simulink model "latLinSim"  (R2021b)
settings: Solver=VariableStepAuto  StartTime=0.0  StopTime=20  RelTol=1e-3
values from neighbouring files (symbols this model uses):
  g = 32.17405    [SingleDOF.m]    (also in layer1atm.m; mainSimple.m = 32.174; simio.m = [dx(Index.EOM(1:6)); delta(:)-f; -delta(:)-f ])
  K_lat_hinf = pss(K_lat_hinfs,Domain)    [SingleDOF.m]    (also in latTest.m; main.m; mainSimple.m; test.m)
  LTI_lat = ss(A_lat,B_lat,C_lat,D_lat)    [Dorobantu.m]    (also in mainLinear.m = GTM_lat(:,:,i,j,k))
libraries: simulink_extras x9
settings Model: Creator=jihoo  LastModifiedBy=jihoo

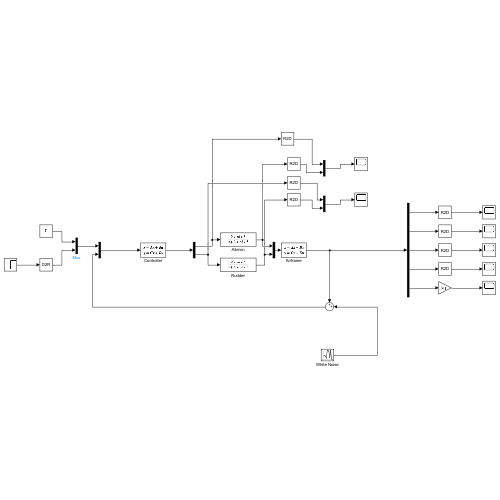
[thumbnail: Simulink's stored preview of the top-level diagram]
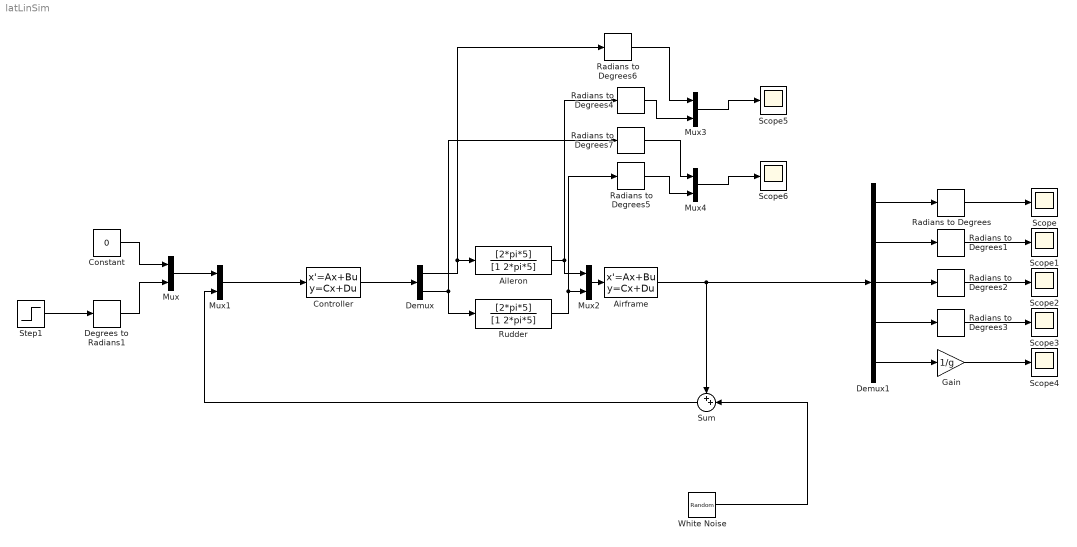
== system latLinSim ==
  Aileron : TransferFcn  Numerator=[2*pi*5]  Denominator=[1 2*pi*5]
  Airframe : StateSpace  A=LTI_lat.A  B=LTI_lat.B  C=LTI_lat.C  D=LTI_lat.D  InitialCondition=0
  Constant : Constant  Value=0
  Controller : StateSpace  A=K_lat_hinf.A  B=K_lat_hinf.B  C=K_lat_hinf.C  D=K_lat_hinf.D  InitialCondition=0
  Degrees to Radians1 : simulink_extras/Transformations/Degrees to Radians
  Demux : Demux  Outputs=2
  Demux1 : Demux  Outputs=5
  Gain : Gain  Gain=1/g
  Mux{,1..4} (5 alike) : Mux  Inputs=2
  Radians to Degrees{,1..7} (8 alike) : simulink_extras/Transformations/Radians to Degrees
  Rudder : TransferFcn  Numerator=[2*pi*5]  Denominator=[1 2*pi*5]
  Scope{,1..6} (7 alike) : Scope
  Step1 : Step  After=45  SampleTime=0
  Sum : Sum  Inputs=++|
  White Noise : RandomNumber  Seed=round(300*rand(1))  SampleTime=1/200
  wires:
  Step1/1 -> Degrees to Radians1/1
  Constant/1 -> Mux/1
  Degrees to Radians1/1 -> Mux/2
  Mux/1 -> Mux1/1
  Mux2/1 -> Airframe/1
  Aileron/1 -> Mux2/1, Radians to Degrees4/1
  Rudder/1 -> Radians to Degrees5/1, Mux2/2
  Mux1/1 -> Controller/1
  Controller/1 -> Demux/1
  Demux/2 -> Rudder/1, Radians to Degrees7/1
  Airframe/1 -> Demux1/1, Sum/1
  Demux1/1 -> Radians to Degrees/1
  Demux1/2 -> Radians to Degrees1/1
  Demux1/3 -> Radians to Degrees2/1
  Demux1/4 -> Radians to Degrees3/1
  Demux1/5 -> Gain/1
  Radians to Degrees/1 -> Scope/1
  Radians to Degrees1/1 -> Scope1/1
  Radians to Degrees2/1 -> Scope2/1
  Radians to Degrees3/1 -> Scope3/1
  Gain/1 -> Scope4/1
  Radians to Degrees6/1 -> Mux3/1
  Demux/1 -> Radians to Degrees6/1, Aileron/1
  Mux3/1 -> Scope5/1
  Radians to Degrees4/1 -> Mux3/2
  Mux4/1 -> Scope6/1
  Radians to Degrees5/1 -> Mux4/2
  Radians to Degrees7/1 -> Mux4/1
  White Noise/1 -> Sum/2
  Sum/1 -> Mux1/2
